simulink model "EV_Subsystem"  (R2024b)
settings: Solver=ode14x  StartTime=0.0  StopTime=2  FixedStep=1e-5  RelTol=1e-3
libraries: spsSeriesRLCBranchLib x4, spsControlledCurrentSourceLib x1, spsCurrentMeasurementLib x1, spsVoltageMeasurementLib x1, spspowerguiLib x1
settings Model: Creator=Raju  LastModifiedBy=Raju

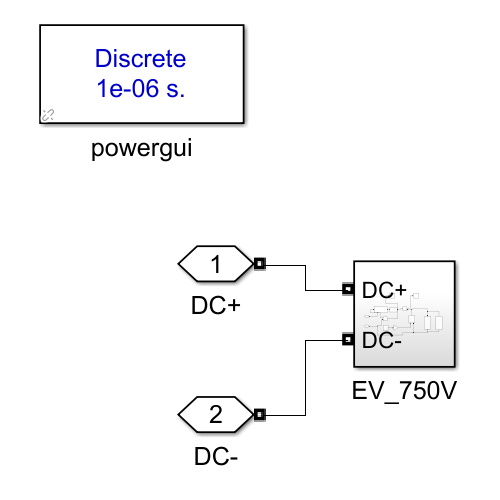
[thumbnail: Simulink's stored preview of the top-level diagram]
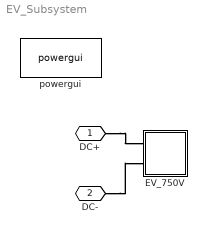
== system EV_Subsystem ==
  EV_750V : Subsystem
  powergui : spspowerguiLib/powergui  Priority=1  SimulationMode=Discrete  SampleTime=1e-6  frequency=60  Iterations=50  frequencyindice=0  Pbase=100e6  ErrMax=1e-4  UnitsV=kV  UnitsW=MW  buscounter=0  FunctionMessages=off  echomessages=off  EnableUseOfTLC=off  CurrentSourceSwitches=off  DisableSnubberDevices=off  DisableRonSwitches=off  DisableVfSwitches=off  DisplayEquations=off  AutomaticDiscreteSolvers=off  SolverType=Tustin/Backward Euler (TBE)  Interpol=off  ExternalGateDelay=off  methode=off  Ts=100  x0status=blocks  SPID=on  SwTol=0  HookPort=off  NonlinearTolerance=1e-4  nMaxIteration=100  ContinueOnMaxIteration=off  RestoreLinks=warning  ResistiveCurrentMeasurement=off  Frange=[0:2:500]  Ylog=off  Xlog=on  ShowGrid=off  save=off  variable=ZData  structure=0  ZoomFFT=off  StartTime=0.0  cycles=1  DisplayStyle=1  fundamental=60  FreqAxis=off  MaxFrequency=1000  frequencyindicesteady=1  RmsSteady=1  display=off
  DC+ : PMIOPort  Side=Left
  DC- : PMIOPort  Port=2  Side=Left
  connections:
  DC+/RConn1 -- EV_750V/LConn1
  DC-/RConn1 -- EV_750V/LConn2

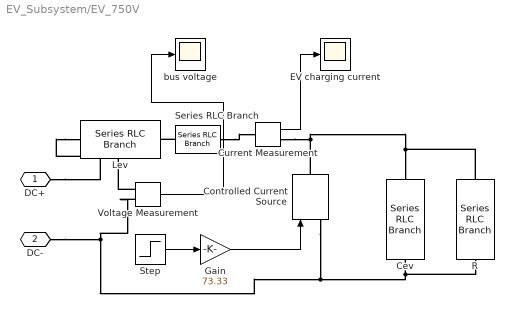
== system EV_Subsystem/EV_750V ==
  Cev : spsSeriesRLCBranchLib/Series RLC Branch  LConnTagsString=__new0  RConnTagsString=__new0  BranchType=C  Resistance=1  Inductance=1e-3  SetiL0=off  InitialCurrent=0  Capacitance=500e-6  Setx0=off  InitialVoltage=0  Measurements=None
  Controlled Current Source : spsControlledCurrentSourceLib/Controlled Current Source  Initialize=on  Source_Type=AC  Amplitude=0  Phase=0  Frequency=0  Measurements=None
  Current Measurement : spsCurrentMeasurementLib/Current Measurement  PhasorSimulation=off  OutputType=Complex  PSBequivalent=0
  EV charging current : Scope
  Gain : Gain  Gain=73.33
  Lev : spsSeriesRLCBranchLib/Series RLC Branch  LConnTagsString=__new0  RConnTagsString=__new0  BranchType=L  Resistance=1  Inductance=2.55e-3  SetiL0=off  InitialCurrent=0  Capacitance=1e-6  Setx0=off  InitialVoltage=0  Measurements=None
  R : spsSeriesRLCBranchLib/Series RLC Branch  LConnTagsString=__new0  RConnTagsString=__new0  BranchType=R  Resistance=1e5  Inductance=1e-3  SetiL0=off  InitialCurrent=0  Capacitance=1e-6  Setx0=off  InitialVoltage=0  Measurements=None
  Series RLC Branch : spsSeriesRLCBranchLib/Series RLC Branch  LConnTagsString=__new0  RConnTagsString=__new0  BranchType=R  Resistance=0.1  Inductance=1e-3  SetiL0=off  InitialCurrent=0  Capacitance=1e-6  Setx0=off  InitialVoltage=0  Measurements=None
  Step : Step  Time=0.2  SampleTime=0
  Voltage Measurement : spsVoltageMeasurementLib/Voltage Measurement  PhasorSimulation=off  OutputType=Complex  PSBequivalent=0
  bus voltage : Scope
  DC+ : PMIOPort  Side=Left
  DC- : PMIOPort  Port=2  Side=Left
  wires:
  Step/1 -> Gain/1
  Gain/1 -> Controlled Current Source/1
  Voltage Measurement/1 -> bus voltage/1
  Current Measurement/1 -> EV charging current/1
  connections:
  Lev/LConn1 -- DC+/RConn1 -- Voltage Measurement/LConn1
  Controlled Current Source/LConn1 -- DC-/RConn1 -- Voltage Measurement/LConn2 -- R/RConn1 -- Cev/RConn1
  Controlled Current Source/RConn1 -- R/LConn1 -- Cev/LConn1 -- Current Measurement/RConn1
  Series RLC Branch/LConn1 -- Lev/RConn1
  Series RLC Branch/RConn1 -- Current Measurement/LConn1
